simulink model "mpc1_1_sansPerturbations"  (R2023a)
settings: Solver=FixedStepDiscrete  StartTime=0.0  StopTime=100  FixedStep=0.5  RelTol=1e-3
libraries: mpclib x1, cstblocks x1
settings Model: Creator=z92504194  LastModifiedBy=z92504194

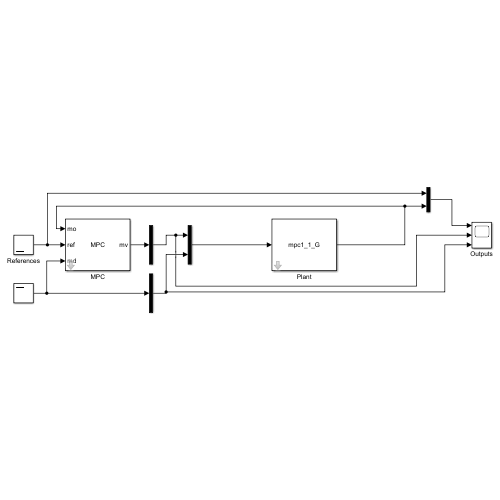
[thumbnail: Simulink's stored preview of the top-level diagram]
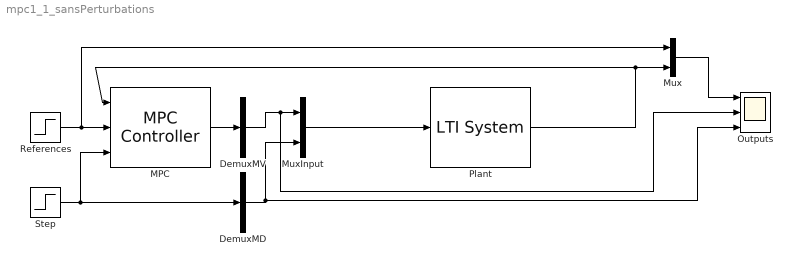
== system mpc1_1_sansPerturbations ==
  DemuxMD : Demux  Outputs=1
  DemuxMV : Demux  Outputs=1
  MPC : mpclib/MPC Controller  SCDEnableBlockLinearizationSpecification=on  mpcobj=mpc1_1_C  is_multiple=0  enable_value=0  return_u0=off  updateMPCinCallerWorkspace=on  md_inport=on  mv_inport=off  uref_inport=off  return_cost=off  return_mvseq=off  return_qpstatus=off  return_xseq=off  return_state=off  return_ovseq=off  state_inport=off  umin_inport=off  umax_inport=off  ymin_inport=off  ymax_inport=off  cc_inport=off  ywt_inport=off  uwt_inport=off  duwt_inport=off  rhoeps_inport=off  pm_inport=off  MaximumP=10  HorizonChoice=FixedHorizon  n_ts=0.5  n_p=10  n_mv=1  n_md=1  n_ud=0  n_mo=1  n_uo=0  BlockDataType=double  SampleTimeInherited=off  switch_inport=off
  Mux : Mux  Inputs=2
  MuxInput : Mux  Inputs=2
  Outputs : Scope  NumInputPorts=3
  Plant : cstblocks/LTI System  sys=mpc1_1_G  IC=[]
  References : Step  Time=10  After=20
  Step : Step  Time=20  After=-5  SampleTime=0
  wires:
  References/1 -> Mux/1, MPC/2
  MuxInput/1 -> Plant/1
  MPC/1 -> DemuxMV/1
  DemuxMV/1 -> Outputs/2, MuxInput/1
  Step/1 -> MPC/3, DemuxMD/1
  DemuxMD/1 -> Outputs/3, MuxInput/2
  Plant/1 -> Mux/2, MPC/1
  Mux/1 -> Outputs/1
